simulink model "nms_sim_2D_cost"  (R2024b)
settings: Solver=ode15s  StartTime=0.0  StopTime=t_sim  MaxStep=dt_max  EnableMultiTasking=on
values from neighbouring files (symbols this model uses):
  a_BFSH = param_ctrl(35)*1    [setCtrlPar_optim_CPGreflex2001_2D.m]
  a_GAS = param_ctrl(37)*1    [setCtrlPar_optim_CPGreflex2001_2D.m]
  a_GLU = param_ctrl(31)*1    [setCtrlPar_optim_CPGreflex2001_2D.m]
  a_HAM = param_ctrl(33)*1    [setCtrlPar_optim_CPGreflex2001_2D.m]
  a_HFL = param_ctrl(32)*1    [setCtrlPar_optim_CPGreflex2001_2D.m]
  a_RF = param_ctrl(34)*1    [setCtrlPar_optim_CPGreflex2001_2D.m]
  a_SOL = param_ctrl(38)*1    [setCtrlPar_optim_CPGreflex2001_2D.m]
  a_TA = param_ctrl(39)*1    [setCtrlPar_optim_CPGreflex2001_2D.m]
  a_VAS = param_ctrl(36)*1    [setCtrlPar_optim_CPGreflex2001_2D.m]
  ai = param_ctrl(96)*2.0    [setCtrlPar_optim_CPGreflex2001_2D.m]
  b_BFSH = param_ctrl(52)*.51    [setCtrlPar_optim_CPGreflex2001_2D.m]
  b_BFSHGAS = param_ctrl(55)*.51    [setCtrlPar_optim_CPGreflex2001_2D.m]
  b_BFSHHAM = param_ctrl(54)*.51    [setCtrlPar_optim_CPGreflex2001_2D.m]
  b_BFSHVAS = param_ctrl(53)*.51    [setCtrlPar_optim_CPGreflex2001_2D.m]
  b_GAS = param_ctrl(59)*.51    [setCtrlPar_optim_CPGreflex2001_2D.m]
  b_GASBFSH = param_ctrl(60)*.51    [setCtrlPar_optim_CPGreflex2001_2D.m]
  b_GASSOL = param_ctrl(61)*.51    [setCtrlPar_optim_CPGreflex2001_2D.m]
  b_GLU = param_ctrl(40)*.51    [setCtrlPar_optim_CPGreflex2001_2D.m]
  b_GLUHAM = param_ctrl(42)*.51    [setCtrlPar_optim_CPGreflex2001_2D.m]
  b_GLUHFL = param_ctrl(41)*.51    [setCtrlPar_optim_CPGreflex2001_2D.m]
  b_HAM = param_ctrl(46)*.51    [setCtrlPar_optim_CPGreflex2001_2D.m]
  b_HAMBFSH = param_ctrl(48)*.51    [setCtrlPar_optim_CPGreflex2001_2D.m]
  b_HAMGLU = param_ctrl(47)*.51    [setCtrlPar_optim_CPGreflex2001_2D.m]
  b_HFL = param_ctrl(43)*.51    [setCtrlPar_optim_CPGreflex2001_2D.m]
  b_HFLGLU = param_ctrl(44)*.51    [setCtrlPar_optim_CPGreflex2001_2D.m]
  b_HFLRF = param_ctrl(45)*.51    [setCtrlPar_optim_CPGreflex2001_2D.m]
  b_RF = param_ctrl(49)*.51    [setCtrlPar_optim_CPGreflex2001_2D.m]
  b_RFHFL = param_ctrl(50)*.51    [setCtrlPar_optim_CPGreflex2001_2D.m]
  b_RFVAS = param_ctrl(51)*.51    [setCtrlPar_optim_CPGreflex2001_2D.m]
  b_SOL = param_ctrl(62)*.51    [setCtrlPar_optim_CPGreflex2001_2D.m]
  b_SOLGAS = param_ctrl(64)*.51    [setCtrlPar_optim_CPGreflex2001_2D.m]
  b_SOLTA = param_ctrl(63)*.51    [setCtrlPar_optim_CPGreflex2001_2D.m]
  b_TA = param_ctrl(65)*.51    [setCtrlPar_optim_CPGreflex2001_2D.m]
  b_TASOL = param_ctrl(66)*.51    [setCtrlPar_optim_CPGreflex2001_2D.m]
  b_VAS = param_ctrl(56)*.51    [setCtrlPar_optim_CPGreflex2001_2D.m]
  b_VASBFSH = param_ctrl(57)*.51    [setCtrlPar_optim_CPGreflex2001_2D.m]
  b_VASRF = param_ctrl(58)*.51    [setCtrlPar_optim_CPGreflex2001_2D.m]
  bias = param_ctrl(97)*2.5    [setCtrlPar_optim_CPGreflex2001_2D.m]
  c = 0.05    [nms_MS_2D_scaled.m]
  c_jointstop = 0.3 / (pi/180)    (= 17.1887338539)    [nms_MS_2D_scaled.m]
  D12_F = 0.16    *scaleL_JPhys    [nms_MechInit_2D_scaleSkel.m]
  D12_S = 0.2460	*sub_height    [nms_MechInit_2D_scaleSkel.m]
  D12_T = 0.2450  *sub_height    [nms_MechInit_2D_scaleSkel.m]
  D12y_F = 0.039  *sub_height    [nms_MechInit_2D_scaleSkel.m]
  D12z_HAT = 0.1    [nms_MS_2D_scaled.m]
  D13_F = 0.20    *scaleL_JPhys    [nms_MechInit_2D_scaleSkel.m]
  D1G_F = 0.14    *scaleL_JPhys    [nms_MechInit_2D_scaleSkel.m]
  D1G_HAT = 0.35  *scaleL_JPhys    [nms_MechInit_2D_scaleSkel.m]
  D1G_S = (0.3 - D12y_F/4)	*scaleL_JPhys    [nms_MechInit_2D_scaleSkel.m]
  D1G_T = (0.3 - D12y_F/4)	*scaleL_JPhys    [nms_MechInit_2D_scaleSkel.m]
  D1Gy_F = D12y_F*D1G_F/D12_F    (= 0.07)    [nms_MechInit_2D_scaleSkel.m]
  d_BFSH = param_ctrl(26)*1    [setCtrlPar_optim_CPGreflex2001_2D.m]
  d_GAS = param_ctrl(28)*1    [setCtrlPar_optim_CPGreflex2001_2D.m]
  d_GLU = param_ctrl(22)*1    [setCtrlPar_optim_CPGreflex2001_2D.m]
  d_HAM = param_ctrl(24)*1    [setCtrlPar_optim_CPGreflex2001_2D.m]
  d_HFL = param_ctrl(23)*1    [setCtrlPar_optim_CPGreflex2001_2D.m]
  d_RF = param_ctrl(25)*1    [setCtrlPar_optim_CPGreflex2001_2D.m]
  d_SOL = param_ctrl(29)*1    [setCtrlPar_optim_CPGreflex2001_2D.m]
  d_TA = param_ctrl(30)*1    [setCtrlPar_optim_CPGreflex2001_2D.m]
  d_VAS = param_ctrl(27)*1    [setCtrlPar_optim_CPGreflex2001_2D.m]
  DeltaThRef = 5e-3    (= 0.005)    [nms_MS_2D_scaled.m]
  dloptBFSH = 3.0    (= 3)    [setCtrlPar_optim_CPGreflex2001_2D.m]
  dloptGAS = 3.0    (= 3)    [setCtrlPar_optim_CPGreflex2001_2D.m]
  dloptGLU = 3.0    (= 3)    [setCtrlPar_optim_CPGreflex2001_2D.m]
  dloptHAM = 3.0    (= 3)    [setCtrlPar_optim_CPGreflex2001_2D.m]
  dloptHFL = 3.0    (= 3)    [setCtrlPar_optim_CPGreflex2001_2D.m]
  dloptRF = 3.0    (= 3)    [setCtrlPar_optim_CPGreflex2001_2D.m]
  dloptSOL = 3.0    (= 3)    [setCtrlPar_optim_CPGreflex2001_2D.m]
  dloptTA = 3.0    (= 3)    [setCtrlPar_optim_CPGreflex2001_2D.m]
  dloptVAS = 3.0    (= 3)    [setCtrlPar_optim_CPGreflex2001_2D.m]
  ec_BFSH = param_ctrl(80)*0.15    [setCtrlPar_optim_CPGreflex2001_2D.m]
  ec_GAS = param_ctrl(82)*0.15    [setCtrlPar_optim_CPGreflex2001_2D.m]
  ec_GLU = param_ctrl(76)*0.15    [setCtrlPar_optim_CPGreflex2001_2D.m]
  ec_HAM = param_ctrl(78)*0.15    [setCtrlPar_optim_CPGreflex2001_2D.m]
  ec_HFL = param_ctrl(77)*0.15    [setCtrlPar_optim_CPGreflex2001_2D.m]
  ec_RF = param_ctrl(79)*0.15    [setCtrlPar_optim_CPGreflex2001_2D.m]
  ec_TA = param_ctrl(84)*0.15    [setCtrlPar_optim_CPGreflex2001_2D.m]
  ec_VAS = param_ctrl(81)*0.15    [setCtrlPar_optim_CPGreflex2001_2D.m]
  eref = 0.04    [nms_MS_2D_scaled.m]
  eref_GAS = 0.1    [nms_MS_2D_scaled.m]
  eref_SOL = 0.1    [nms_MS_2D_scaled.m]
  es_BFSH = param_ctrl(89)*0.15    [setCtrlPar_optim_CPGreflex2001_2D.m]
  es_GAS = param_ctrl(91)*0.15    [setCtrlPar_optim_CPGreflex2001_2D.m]
  es_GLU = param_ctrl(85)*0.15    [setCtrlPar_optim_CPGreflex2001_2D.m]
  es_HAM = param_ctrl(87)*0.15    [setCtrlPar_optim_CPGreflex2001_2D.m]
  es_HFL = param_ctrl(86)*0.15    [setCtrlPar_optim_CPGreflex2001_2D.m]
  es_RF = param_ctrl(88)*0.15    [setCtrlPar_optim_CPGreflex2001_2D.m]
  es_TA = param_ctrl(93)*0.15    [setCtrlPar_optim_CPGreflex2001_2D.m]
  es_VAS = param_ctrl(90)*0.15    [setCtrlPar_optim_CPGreflex2001_2D.m]
  FmaxBFSH = 350    [nms_MS_2D_scaled.m]
  FmaxGAS = 2000    [nms_MS_2D_scaled.m]
  FmaxGLU = 4000    [nms_MS_2D_scaled.m]
  FmaxHAM = 2000    [nms_MS_2D_scaled.m]
  FmaxHFL = 2000    [nms_MS_2D_scaled.m]
  FmaxRF = 850    [nms_MS_2D_scaled.m]
  FmaxSOL = 4000    [nms_MS_2D_scaled.m]
  FmaxTA = 800    [nms_MS_2D_scaled.m]
  FmaxVAS = 5000    [nms_MS_2D_scaled.m]
  g = 9.81    [nms_MS_2D_scaled.m]
  gamma_4 = param_ctrl(11) * 1.7    [setCtrlPar_optim_CPGreflexsynergy2023_2D.m]
  h_BFSH = param_ctrl(71)*.1    [setCtrlPar_optim_CPGreflex2001_2D.m]
  h_GAS = param_ctrl(73)*.1    [setCtrlPar_optim_CPGreflex2001_2D.m]
  h_GLU = param_ctrl(67)*.1    [setCtrlPar_optim_CPGreflex2001_2D.m]
  h_HAM = param_ctrl(69)*.1    [setCtrlPar_optim_CPGreflex2001_2D.m]
  h_HFL = param_ctrl(68)*.1    [setCtrlPar_optim_CPGreflex2001_2D.m]
  h_RF = param_ctrl(70)*.1    [setCtrlPar_optim_CPGreflex2001_2D.m]
  h_SOL = param_ctrl(74)*.1    [setCtrlPar_optim_CPGreflex2001_2D.m]
  h_TA = param_ctrl(75)*.1    [setCtrlPar_optim_CPGreflex2001_2D.m]
  h_VAS = param_ctrl(72)*.1    [setCtrlPar_optim_CPGreflex2001_2D.m]
  HLCtrlPar = [theta_tgt l_clr alpha_tgt alpha_cd alpha_cv]    [setCtrlPar_optim_reflex2015_2D.m]
  In_F = 0.005    *scaleM*scaleL_JPhys^2    [nms_MechInit_2D_scaleSkel.m]
  In_HAT = 2.5    *scaleM*scaleL_JPhys^2    [nms_MechInit_2D_scaleSkel.m]
  In_S = 0.05     *scaleM*scaleL_JPhys^2    [nms_MechInit_2D_scaleSkel.m]
  In_T = 0.15     *scaleM*scaleL_JPhys^2    [nms_MechInit_2D_scaleSkel.m]
  init_exc = 0.01    [setInitPar_optim_2D.m]
  init_fm = 0.01    [setInitPar_optim_2D.m]
  init_lce = 1    [setInitPar_optim_2D.m]
  init_LCPG = param_ctrl(12) * 0.01    [setCtrlPar_optim_CPGreflexsynergy2023_2D.m]
  init_LStance = 1    [setInitPar_optim_2D.m]
  init_N1 = osc_signal1(phi_off_osc_ind)    [setCtrlPar_optim_CPGreflex2001_2D.m]
  ... (+441 more)
undefined symbols (not defined in the file or in its folder): cost_act_exponent, cost_v_tgt, flag_controller, Newton, nStep_obj, nStep_startKin, Raphson, sgn, SSW_kin, terrain_slope_angle, v_plateS1, X, Y, Z
libraries: nesl_utility x94, sm_lib x90, simulink x28, simulink_extras x12
(part 1 of 20)
settings Model: SimulationMode=accelerator  Creator=smsong  LastModifiedBy=tonvi
settings SolverCC: ZeroCrossControl=DisableAll  AlgebraicLoopSolver=TrustRegion
settings DataIOCC: LimitDataPoints=on  SaveFormat=Array  SaveOutput=off  SignalLogging=off  DSMLogging=off  SaveTime=off
settings OptimizationCC: BooleanDataType=off  ReuseModelBlockBuffer=off  LifeSpan=inf
settings DebuggingCC: UnconnectedInputMsg=warning  UnconnectedOutputMsg=warning  UnconnectedLineMsg=warning  SFUnexpectedBacktrackingDiag=warning  SFNoUnconditionalDefaultTransitionDiag=warning  SFExecutionAtInitializationDiag=none  ArithmeticOperatorsInVariantConditions=warning
settings HardwareCC: ProdBitPerPointer=32  ProdBitPerSizeT=32  ProdBitPerPtrDiffT=32  ProdLargestAtomicFloat=None  ProdIntDivRoundTo=Undefined  ProdEndianess=Unspecified  ProdWordSize=32  ProdHWDeviceType=32-bit Generic
settings ModelReferenceCC: EnableRefExpFcnMdlSchedulingChecks=on  PropagateSignalLabelsOutOfModel=off
settings SFSimCC: SimUseLocalCustomCode=off  CustomCodeUndefinedFunction=UseInterfaceOnly
settings RTWCC: RTWUseLocalCustomCode=off  GPUComputeCapability=3.5
settings CodeAppCC: StateflowObjectComments=on
settings GRTTargetCC: TargetLangStandard=C89/C90 (ANSI)
settings ConfigComp: CovMetricSettings=dw  CovSaveCumulativeToWorkspaceVar=on  CovSaveSingleToWorkspaceVar=on  CovExternalEMLEnable=off
settings SimscapeCC: SimscapeNormalizeSystem=off
settings ConfigurationSet: Description=SimMechanics 2G
settings ExplorerConfigSet: InternalSimMechanicsExplorerSettings="<ExplorerConfiguration><canonicalview>planar_xy</canonicalview><AnimationSetting><BasePlaybackSpeed>1.0</BasePlaybackSpeed><PlaybackSpeedFactor>1.0</PlaybackSpeedFactor></AnimationSetting><TilePanel><TileInfo><Tiles Columns=\"1\" Count=\"1\" Rows=\"1\"><Column Weight=\"1\"/><Row Weight=\"1\"/><Tile Height=\"1\" Width=\"1\" X=\"0\" Y=\"0\"/></Tiles></TileInfo><SceneInfo><SceneViewer><BGColor><R>1</R><G>1</G><B>1</B></BGColor><Camera><DoPerspective>off</DoPerspective><Position><X>-0.261050130897375665</X><Y>1.42717715276589785</Y><Z>30.2910165948773908</Z></Position><Center><X>-0.261050130897375665</X><Y>1.42717715276589785</Y><Z>-2.94192883387722759e-08</Z></Center><Up><X>0</X><Y>1</Y><Z>0</Z></Up><ViewLimDist>1</ViewLimDist><YLim>2.31502487225703657</YLim><XLim>2.56039617208151515</XLim></Camera></SceneViewer></SceneInfo></TilePanel><MechEditorPanel><Cameras/><GfxPanelCameraMap/><VideoCreator><PlaybackSpeedRatio>1.0</PlaybackSpeedRatio><FrameRate>30</FrameRate><VideoFormat>Motion JPEG AVI</VideoFormat><FrameSize>auto</FrameSize></VideoCreator></MechEditorPanel></ExplorerConfiguration>"

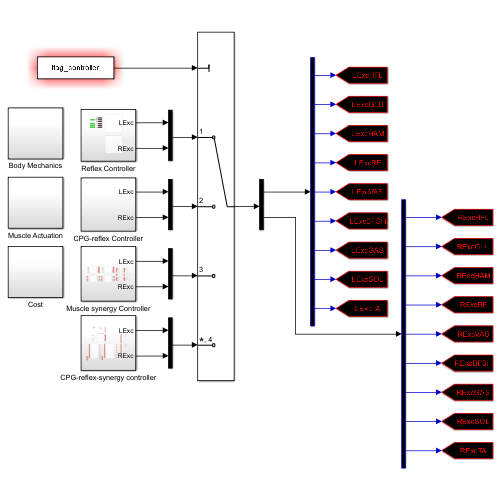
[thumbnail: Simulink's stored preview of the top-level diagram]
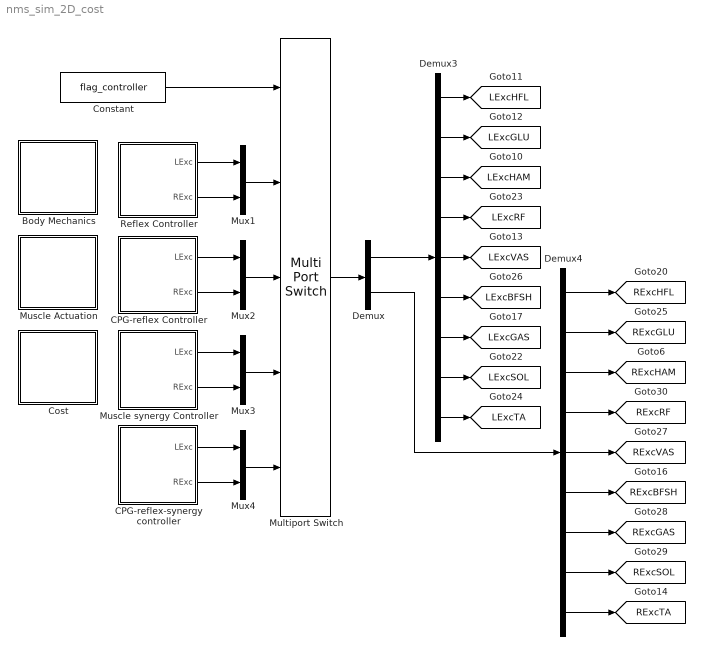
== system nms_sim_2D_cost ==
  Body Mechanics : Subsystem
  CPG-reflex Controller : Subsystem
  CPG-reflex-synergy controller : Subsystem
  Constant : Constant  Value=flag_controller
  Cost : Subsystem
  Demux : Demux  Outputs=2
  Demux3 : Demux  Outputs=9
  Demux4 : Demux  Outputs=9
  Multiport Switch : MultiPortSwitch  Inputs=4  SaturateOnIntegerOverflow=off  InputSameDT=off
  Muscle Actuation : Subsystem
  Muscle synergy Controller : Subsystem
  Mux{1..4} (4 alike) : Mux  Inputs=2
  Reflex Controller : Subsystem
  tag scope: LExcBFSH=global, LExcGAS=global, LExcGLU=global, LExcHAM=global, LExcHFL=global, LExcRF=global, LExcSOL=global, LExcTA=global, LExcVAS=global, RExcBFSH=global, RExcGAS=global, RExcGLU=global, RExcHAM=global, RExcHFL=global, RExcRF=global, RExcSOL=global, RExcTA=global, RExcVAS=global
  wires:
  Demux3/9 -> [LExcTA]
  Demux/1 -> Demux3/1
  Demux3/4 -> [LExcRF]
  Demux3/6 -> [LExcBFSH]
  Demux3/1 -> [LExcHFL]
  Demux3/8 -> [LExcSOL]
  Demux3/3 -> [LExcHAM]
  Demux3/7 -> [LExcGAS]
  Demux3/5 -> [LExcVAS]
  Demux3/2 -> [LExcGLU]
  Demux/2 -> Demux4/1
  Demux4/7 -> [RExcGAS]
  Demux4/8 -> [RExcSOL]
  Demux4/5 -> [RExcVAS]
  Demux4/2 -> [RExcGLU]
  Demux4/4 -> [RExcRF]
  Demux4/3 -> [RExcHAM]
  Demux4/1 -> [RExcHFL]
  Demux4/6 -> [RExcBFSH]
  Demux4/9 -> [RExcTA]
  Constant/1 -> Multiport Switch/1
  Reflex Controller/1(LExc) -> Mux1/1
  Reflex Controller/2(RExc) -> Mux1/2
  CPG-reflex-synergy controller/2(RExc) -> Mux4/2
  CPG-reflex-synergy controller/1(LExc) -> Mux4/1
  Multiport Switch/1 -> Demux/1
  Mux1/1 -> Multiport Switch/2
  Mux4/1 -> Multiport Switch/5
  Muscle synergy Controller/1(LExc) -> Mux3/1
  Muscle synergy Controller/2(RExc) -> Mux3/2
  Mux2/1 -> Multiport Switch/3
  Mux3/1 -> Multiport Switch/4
  CPG-reflex Controller/1(LExc) -> Mux2/1
  CPG-reflex Controller/2(RExc) -> Mux2/2

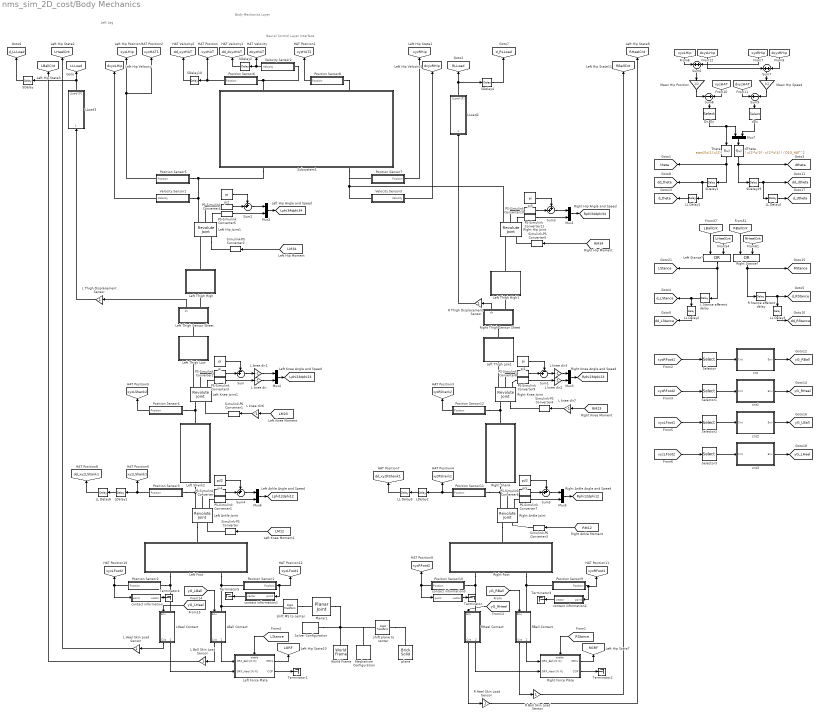
== system nms_sim_2D_cost/Body Mechanics ==
  note: Body Mechanics Layer
  note: Left Leg
  note: Neural Control Layer Interface
  " Mean Hip Speed" : Gain  Gain=1/2
  "Dx, Dy" : Selector  InputPortWidth=3  IndexOptions=Index vector (dialog)  Indices=[1 2]  OutputSizes=1
  L Ball Skin Load Sensor : Gain
  L Heel Skin Load Sensor : Gain
  L Stance afferent delay : TransportDelay  DelayTime=MidDelay  InitialOutput=init_LStance
  L Thigh Displacement  Sensor : Gain
  L knee dir{,1..3,6..7} (6 alike) : Gain  Gain=-1
  LBall Contact : Subsystem
  LDelay1 : TransportDelay  DelayTime=LongDelay  InitialOutput=init_xyzLShank
  LDelay2 : TransportDelay  DelayTime=LongDelay  InitialOutput=init_xyzRShank
  LHeel Contact : Subsystem
  LL Delay1 : TransportDelay  DelayTime=LongLoopDelay  InitialOutput=init_theta
  LL Delay2 : TransportDelay  DelayTime=LongLoopDelay  InitialOutput=init_LStance
  LL Delay3 : TransportDelay  DelayTime=LongLoopDelay  InitialOutput=init_RStance
  LL Delay4 : TransportDelay  DelayTime=LongLoopDelay
  LL Delay5 : TransportDelay  DelayTime=LongLoopDelay  InitialOutput=init_xyzRShank
  LL Delay6 : TransportDelay  DelayTime=LongLoopDelay  InitialOutput=init_xyzLShank
  LLoad2 : Subsystem
  LLoad3 : Subsystem
  Left Ankle Joint : sm_lib/Joints/Revolute Joint  JointMode=Normal  CompositeWrenchDir=FollowerOnBase  CompositeWrenchFrame=BaseFrame  SenseConstraintForce=off  SenseConstraintTorque=off  SenseTotalForce=off  SenseTotalTorque=off  PositionTargetSpecify=on  PositionTargetPriority=High  PositionTargetValue=Lphi120-pi/2  PositionTargetValueUnits=rad  VelocityTargetSpecify=on  VelocityTargetPriority=High  VelocityTargetValue=0  VelocityTargetValueUnits=rad/s  EquilibriumPosition=0  EquilibriumPositionUnits=deg  SpringStiffness=0  SpringStiffnessUnits=N*m/deg  DampingCoefficient=0  DampingCoefficientUnits=N*m/(deg/s)  LowerLimitSpecify=off  LowerLimitBound=-90  LowerLimitBoundUnits=deg  LowerLimitStiffness=1e4  LowerLimitStiffnessUnits=N*m/deg  LowerLimitDamping=10  LowerLimitDampingUnits=N*m/(deg/s)  LowerLimitTransitionRegionWidth=0.1  LowerLimitTransitionRegionWidthUnits=deg  UpperLimitSpecify=off  UpperLimitBound=90  UpperLimitBoundUnits=deg  UpperLimitStiffness=1e4  UpperLimitStiffnessUnits=N*m/deg  UpperLimitDamping=10  UpperLimitDampingUnits=N*m/(deg/s)  UpperLimitTransitionRegionWidth=0.1  UpperLimitTransitionRegionWidthUnits=deg  TorqueActuationMode=InputTorque  MotionActuationMode=ComputedMotion  SensePosition=on  SenseVelocity=on  SenseAcceleration=off  SenseTorqueForce=off  SenseLowerLimitTorqueForce=off  SenseUpperLimitTorqueForce=off
  Left Hip Joint1 : sm_lib/Joints/Revolute Joint  JointMode=Normal  CompositeWrenchDir=FollowerOnBase  CompositeWrenchFrame=BaseFrame  SenseConstraintForce=off  SenseConstraintTorque=off  SenseTotalForce=off  SenseTotalTorque=off  PositionTargetSpecify=on  PositionTargetPriority=High  PositionTargetValue=Lphi340-pi  PositionTargetValueUnits=rad  VelocityTargetSpecify=on  VelocityTargetPriority=High  VelocityTargetValue=0  VelocityTargetValueUnits=rad/s  EquilibriumPosition=0  EquilibriumPositionUnits=deg  SpringStiffness=0  SpringStiffnessUnits=N*m/deg  DampingCoefficient=0  DampingCoefficientUnits=N*m/(deg/s)  LowerLimitSpecify=off  LowerLimitBound=-90  LowerLimitBoundUnits=deg  LowerLimitStiffness=1e4  LowerLimitStiffnessUnits=N*m/deg  LowerLimitDamping=10  LowerLimitDampingUnits=N*m/(deg/s)  LowerLimitTransitionRegionWidth=0.1  LowerLimitTransitionRegionWidthUnits=deg  UpperLimitSpecify=off  UpperLimitBound=90  UpperLimitBoundUnits=deg  UpperLimitStiffness=1e4  UpperLimitStiffnessUnits=N*m/deg  UpperLimitDamping=10  UpperLimitDampingUnits=N*m/(deg/s)  UpperLimitTransitionRegionWidth=0.1  UpperLimitTransitionRegionWidthUnits=deg  TorqueActuationMode=InputTorque  MotionActuationMode=ComputedMotion  SensePosition=on  SenseVelocity=on  SenseAcceleration=off  SenseTorqueForce=off  SenseLowerLimitTorqueForce=off  SenseUpperLimitTorqueForce=off
  Left Knee Joint1 : sm_lib/Joints/Revolute Joint  JointMode=Normal  CompositeWrenchDir=FollowerOnBase  CompositeWrenchFrame=BaseFrame  SenseConstraintForce=off  SenseConstraintTorque=off  SenseTotalForce=off  SenseTotalTorque=off  PositionTargetSpecify=on  PositionTargetPriority=High  PositionTargetValue=pi-Lphi230  PositionTargetValueUnits=rad  VelocityTargetSpecify=on  VelocityTargetPriority=High  VelocityTargetValue=0  VelocityTargetValueUnits=rad/s  EquilibriumPosition=0  EquilibriumPositionUnits=deg  SpringStiffness=0  SpringStiffnessUnits=N*m/deg  DampingCoefficient=0  DampingCoefficientUnits=N*m/(deg/s)  LowerLimitSpecify=off  LowerLimitBound=-90  LowerLimitBoundUnits=deg  LowerLimitStiffness=1e4  LowerLimitStiffnessUnits=N*m/deg  LowerLimitDamping=10  LowerLimitDampingUnits=N*m/(deg/s)  LowerLimitTransitionRegionWidth=0.1  LowerLimitTransitionRegionWidthUnits=deg  UpperLimitSpecify=off  UpperLimitBound=90  UpperLimitBoundUnits=deg  UpperLimitStiffness=1e4  UpperLimitStiffnessUnits=N*m/deg  UpperLimitDamping=10  UpperLimitDampingUnits=N*m/(deg/s)  UpperLimitTransitionRegionWidth=0.1  UpperLimitTransitionRegionWidthUnits=deg  TorqueActuationMode=InputTorque  MotionActuationMode=ComputedMotion  SensePosition=on  SenseVelocity=on  SenseAcceleration=off  SenseTorqueForce=off  SenseLowerLimitTorqueForce=off  SenseUpperLimitTorqueForce=off
  Left Foot : Subsystem
  Left Force Plate : Subsystem  TreatAsAtomicUnit=on
  Left Shank2 : Subsystem
  Left Stance? : Logic  Operator=OR  AllPortsSameDT=off
  Left Thigh Sensor Sheet : Subsystem
  Left Thigh High : Subsystem
  Left Thigh High1 : Subsystem
  Left Thigh Low : Subsystem
  Left Thigh Low1 : Subsystem
  Mean Hip Position : Gain  Gain=1/2
  Mechanism Configuration : sm_lib/Utilities/Mechanism Configuration  UniformGravity=Constant  GravityVector=[0 -g 0]  GravityVectorUnits=m/s^2  LinearizationDelta=0.001  JointModeTransitionNonlinearIterations=2
  Mux{1..7} (7 alike) : Mux  Inputs=2
  PS-Simulink Converter{,2,4,6,8,10} (6 alike) : nesl_utility/PS-Simulink Converter  PhysicalDomain=network_engine_domain  SubClassName=ps_output  LeftPortType=input  RightPortType=output  PseudoPeriodic=off  Frequencies=[]  VectorFormat=1-D array  Unit=rad  AffineConversion=off
  PS-Simulink Converter{1,3,5,7,9,11} (6 alike) : nesl_utility/PS-Simulink Converter  PhysicalDomain=network_engine_domain  SubClassName=ps_output  LeftPortType=input  RightPortType=output  PseudoPeriodic=off  Frequencies=[]  VectorFormat=1-D array  Unit=rad/s  AffineConversion=off
  Planar1 : sm_lib/Joints/Planar Joint  JointMode=Normal  CompositeWrenchDir=FollowerOnBase  CompositeWrenchFrame=BaseFrame  SenseConstraintForce=off  SenseConstraintTorque=off  SenseTotalForce=off  SenseTotalTorque=off  PxPositionTargetSpecify=on  PxPositionTargetPriority=High  PxPositionTargetValue=x0  PxPositionTargetValueUnits=m  PxVelocityTargetSpecify=on  PxVelocityTargetPriority=High  PxVelocityTargetValue=vx0  PxVelocityTargetValueUnits=m/s  PxEquilibriumPosition=0  PxEquilibriumPositionUnits=m  PxSpringStiffness=0  PxSpringStiffnessUnits=N/m  PxDampingCoefficient=0  PxDampingCoefficientUnits=N/(m/s)  PxLowerLimitSpecify=off  PxLowerLimitBound=-1  PxLowerLimitBoundUnits=m  PxLowerLimitStiffness=1e6  PxLowerLimitStiffnessUnits=N/m  PxLowerLimitDamping=1e3  PxLowerLimitDampingUnits=N/(m/s)  PxLowerLimitTransitionRegionWidth=1e-4  PxLowerLimitTransitionRegionWidthUnits=m  PxUpperLimitSpecify=off  PxUpperLimitBound=1  PxUpperLimitBoundUnits=m  PxUpperLimitStiffness=1e6  PxUpperLimitStiffnessUnits=N/m  PxUpperLimitDamping=1e3  PxUpperLimitDampingUnits=N/(m/s)  PxUpperLimitTransitionRegionWidth=1e-4  PxUpperLimitTransitionRegionWidthUnits=m  PxTorqueActuationMode=NoTorque  PxMotionActuationMode=ComputedMotion  PxSensePosition=off  PxSenseVelocity=off  PxSenseAcceleration=off  PxSenseTorqueForce=off  PxSenseLowerLimitTorqueForce=off  PxSenseUpperLimitTorqueForce=off  PyPositionTargetSpecify=on  PyPositionTargetPriority=High  PyPositionTargetValue=y0  PyPositionTargetValueUnits=m  PyVelocityTargetSpecify=on  PyVelocityTargetPriority=High  PyVelocityTargetValue=0  PyVelocityTargetValueUnits=m/s  PyEquilibriumPosition=0  PyEquilibriumPositionUnits=m  PySpringStiffness=0  PySpringStiffnessUnits=N/m  PyDampingCoefficient=0  PyDampingCoefficientUnits=N/(m/s)  PyLowerLimitSpecify=off  PyLowerLimitBound=-1  PyLowerLimitBoundUnits=m  PyLowerLimitStiffness=1e6  PyLowerLimitStiffnessUnits=N/m  PyLowerLimitDamping=1e3  PyLowerLimitDampingUnits=N/(m/s)  PyLowerLimitTransitionRegionWidth=1e-4  PyLowerLimitTransitionRegionWidthUnits=m  PyUpperLimitSpecify=off  PyUpperLimitBound=1  PyUpperLimitBoundUnits=m  PyUpperLimitStiffness=1e6  PyUpperLimitStiffnessUnits=N/m  PyUpperLimitDamping=1e3  PyUpperLimitDampingUnits=N/(m/s)  PyUpperLimitTransitionRegionWidth=1e-4  PyUpperLimitTransitionRegionWidthUnits=m  PyTorqueActuationMode=NoTorque  PyMotionActuationMode=ComputedMotion  PySensePosition=off  PySenseVelocity=off  PySenseAcceleration=off  PySenseTorqueForce=off  PySenseLowerLimitTorqueForce=off  PySenseUpperLimitTorqueForce=off  RzPositionTargetSpecify=on  RzPositionTargetPriority=High  RzPositionTargetValue=phi0  RzPositionTargetValueUnits=rad  RzVelocityTargetSpecify=on  RzVelocityTargetPriority=High  RzVelocityTargetValue=0  RzVelocityTargetValueUnits=rad/s  RzEquilibriumPosition=0  RzEquilibriumPositionUnits=deg  RzSpringStiffness=0  RzSpringStiffnessUnits=N*m/deg  RzDampingCoefficient=0  RzDampingCoefficientUnits=N*m/(deg/s)  RzLowerLimitSpecify=off  RzLowerLimitBound=-90  RzLowerLimitBoundUnits=deg  RzLowerLimitStiffness=1e4  RzLowerLimitStiffnessUnits=N*m/deg  RzLowerLimitDamping=10  RzLowerLimitDampingUnits=N*m/(deg/s)  RzLowerLimitTransitionRegionWidth=0.1  RzLowerLimitTransitionRegionWidthUnits=deg  RzUpperLimitSpecify=off  RzUpperLimitBound=90  RzUpperLimitBoundUnits=deg  RzUpperLimitStiffness=1e4  RzUpperLimitStiffnessUnits=N*m/deg  RzUpperLimitDamping=10  RzUpperLimitDampingUnits=N*m/(deg/s)  RzUpperLimitTransitionRegionWidth=0.1  RzUpperLimitTransitionRegionWidthUnits=deg  RzTorqueActuationMode=NoTorque  RzMotionActuationMode=ComputedMotion  RzSensePosition=off  RzSenseVelocity=off  RzSenseAcceleration=off  RzSenseTorqueForce=off  RzSenseLowerLimitTorqueForce=off  RzSenseUpperLimitTorqueForce=off
  Position Sensor1 : Subsystem
  Position Sensor10 : Subsystem
  Position Sensor11 : Subsystem
  Position Sensor12 : Subsystem
  Position Sensor2 : Subsystem
  Position Sensor3 : Subsystem
  Position Sensor4 : Subsystem
  Position Sensor5 : Subsystem
  Position Sensor6 : Subsystem
  Position Sensor7 : Subsystem
  Position Sensor8 : Subsystem
  Position Sensor9 : Subsystem
  R Ball Skin Load Sensor : Gain
  R Heel Skin Load Sensor : Gain
  R Stance afferent delay : TransportDelay  DelayTime=MidDelay  InitialOutput=init_RStance
  R Thigh Displacement  Sensor : Gain
  RBall Contact : Subsystem
  RHeel Contact : Subsystem
  Right Ankle Joint : sm_lib/Joints/Revolute Joint  JointMode=Normal  CompositeWrenchDir=FollowerOnBase  CompositeWrenchFrame=BaseFrame  SenseConstraintForce=off  SenseConstraintTorque=off  SenseTotalForce=off  SenseTotalTorque=off  PositionTargetSpecify=on  PositionTargetPriority=High  PositionTargetValue=Rphi120-pi/2  PositionTargetValueUnits=rad  VelocityTargetSpecify=on  VelocityTargetPriority=High  VelocityTargetValue=0  VelocityTargetValueUnits=rad/s  EquilibriumPosition=0  EquilibriumPositionUnits=deg  SpringStiffness=0  SpringStiffnessUnits=N*m/deg  DampingCoefficient=0  DampingCoefficientUnits=N*m/(deg/s)  LowerLimitSpecify=off  LowerLimitBound=-90  LowerLimitBoundUnits=deg  LowerLimitStiffness=1e4  LowerLimitStiffnessUnits=N*m/deg  LowerLimitDamping=10  LowerLimitDampingUnits=N*m/(deg/s)  LowerLimitTransitionRegionWidth=0.1  LowerLimitTransitionRegionWidthUnits=deg  UpperLimitSpecify=off  UpperLimitBound=90  UpperLimitBoundUnits=deg  UpperLimitStiffness=1e4  UpperLimitStiffnessUnits=N*m/deg  UpperLimitDamping=10  UpperLimitDampingUnits=N*m/(deg/s)  UpperLimitTransitionRegionWidth=0.1  UpperLimitTransitionRegionWidthUnits=deg  TorqueActuationMode=InputTorque  MotionActuationMode=ComputedMotion  SensePosition=on  SenseVelocity=on  SenseAcceleration=off  SenseTorqueForce=off  SenseLowerLimitTorqueForce=off  SenseUpperLimitTorqueForce=off
  Right Hip Joint : sm_lib/Joints/Revolute Joint  JointMode=Normal  CompositeWrenchDir=FollowerOnBase  CompositeWrenchFrame=BaseFrame  SenseConstraintForce=off  SenseConstraintTorque=off  SenseTotalForce=off  SenseTotalTorque=off  PositionTargetSpecify=on  PositionTargetPriority=High  PositionTargetValue=Rphi340-pi  PositionTargetValueUnits=rad  VelocityTargetSpecify=on  VelocityTargetPriority=High  VelocityTargetValue=0  VelocityTargetValueUnits=rad/s  EquilibriumPosition=0  EquilibriumPositionUnits=deg  SpringStiffness=0  SpringStiffnessUnits=N*m/deg  DampingCoefficient=0  DampingCoefficientUnits=N*m/(deg/s)  LowerLimitSpecify=off  LowerLimitBound=-90  LowerLimitBoundUnits=deg  LowerLimitStiffness=1e4  LowerLimitStiffnessUnits=N*m/deg  LowerLimitDamping=10  LowerLimitDampingUnits=N*m/(deg/s)  LowerLimitTransitionRegionWidth=0.1  LowerLimitTransitionRegionWidthUnits=deg  UpperLimitSpecify=off  UpperLimitBound=90  UpperLimitBoundUnits=deg  UpperLimitStiffness=1e4  UpperLimitStiffnessUnits=N*m/deg  UpperLimitDamping=10  UpperLimitDampingUnits=N*m/(deg/s)  UpperLimitTransitionRegionWidth=0.1  UpperLimitTransitionRegionWidthUnits=deg  TorqueActuationMode=InputTorque  MotionActuationMode=ComputedMotion  SensePosition=on  SenseVelocity=on  SenseAcceleration=off  SenseTorqueForce=off  SenseLowerLimitTorqueForce=off  SenseUpperLimitTorqueForce=off
  Right Knee Joint : sm_lib/Joints/Revolute Joint  JointMode=Normal  CompositeWrenchDir=FollowerOnBase  CompositeWrenchFrame=BaseFrame  SenseConstraintForce=off  SenseConstraintTorque=off  SenseTotalForce=off  SenseTotalTorque=off  PositionTargetSpecify=on  PositionTargetPriority=High  PositionTargetValue=pi-Rphi230  PositionTargetValueUnits=rad  VelocityTargetSpecify=on  VelocityTargetPriority=High  VelocityTargetValue=0  VelocityTargetValueUnits=rad/s  EquilibriumPosition=0  EquilibriumPositionUnits=deg  SpringStiffness=0  SpringStiffnessUnits=N*m/deg  DampingCoefficient=0  DampingCoefficientUnits=N*m/(deg/s)  LowerLimitSpecify=off  LowerLimitBound=-90  LowerLimitBoundUnits=deg  LowerLimitStiffness=1e4  LowerLimitStiffnessUnits=N*m/deg  LowerLimitDamping=10  LowerLimitDampingUnits=N*m/(deg/s)  LowerLimitTransitionRegionWidth=0.1  LowerLimitTransitionRegionWidthUnits=deg  UpperLimitSpecify=off  UpperLimitBound=90  UpperLimitBoundUnits=deg  UpperLimitStiffness=1e4  UpperLimitStiffnessUnits=N*m/deg  UpperLimitDamping=10  UpperLimitDampingUnits=N*m/(deg/s)  UpperLimitTransitionRegionWidth=0.1  UpperLimitTransitionRegionWidthUnits=deg  TorqueActuationMode=InputTorque  MotionActuationMode=ComputedMotion  SensePosition=on  SenseVelocity=on  SenseAcceleration=off  SenseTorqueForce=off  SenseLowerLimitTorqueForce=off  SenseUpperLimitTorqueForce=off
  Right Foot : Subsystem
  Right Force Plate : Subsystem  TreatAsAtomicUnit=on
  Right Shank : Subsystem
  Right Stance? : Logic  Operator=OR  AllPortsSameDT=off
  Right Thigh Sensor Sheet : Subsystem
  SDelay : TransportDelay  DelayTime=ShortDelay
  SDelay1 : TransportDelay  DelayTime=ShortDelay  InitialOutput=init_theta
  SDelay10 : TransportDelay  DelayTime=ShortDelay  InitialOutput=init_xyzHAT
  SDelay2 : TransportDelay  DelayTime=ShortDelay  InitialOutput=[vx0 0 0]
  SDelay29 : TransportDelay  DelayTime=ShortDelay
  SDelay4 : TransportDelay  DelayTime=ShortDelay
  Selector{,1..3} (4 alike) : Selector  InputPortWidth=3  IndexOptions=Index vector (dialog)  Indices=[1 2]  OutputSizes=1
  Simulink-PS Converter{,1..5} (6 alike) : nesl_utility/Simulink-PS Converter  PhysicalDomain=network_engine_domain  SubClassName=ps_input  LeftPortType=input  RightPortType=output  PseudoPeriodic=off  Frequencies=[]  NoiseDistribution=none  NoiseParameters=[]  Unit=N*m  AffineConversion=off  FilteringAndDerivatives=zero  SimscapeFilterOrder=1  InputFilterTimeConstant=0.001  UdotUserProvided=1
  Solver Configuration : nesl_utility/Solver Configuration  PhysicalDomain=network_engine_domain  SubClassName=solver  LeftPortType=input  RightPortType=generic  Tones=[]  Harmonics=[]  SimulateNoise=off  Profile=off  UseLocalSampling=off  EnableSwitchedLinearOptims=on  FrequencyDomain=off  UseCCode=off  RelTol=0.001  AbsTol=1e-06  MinStep=1e-09  ToWorkspace=off  RevertToSquareIcSolve=off  NumHomotopyIterations=100  PhasorMode=off  PhasorModeNumHarmonics=1  ConsistencySolver=NEWTON_FTOL  IndexReductionMethod=DerivativeReplacement  DoDC=off  ResidualTolerance=1e-09  ConsistencyTolSource=GLOBAL  ConsistencyAbsTol=0.001  ConsistencyRelTol=0.001  ConsistencyTolFactor=0.001  UseLocalSolver=off  LocalSolverChoice=NE_BACKWARD_EULER_ADVANCER  ResolveIndetEquations=on  FunctionEvalNumThread=1  LocalSolverSampleTime=0.001  DoFixedCost=off  MaxNonlinIter=3  MaxModeIter=2  ComputeImpulses=off  ImpulseIterations=2  LinearAlgebra=Sparse  LinearAlgebraNumThread=0  EquationFormulation=NE_TIME_EF  DelaysMemoryBudget=1024  AutomaticFiltering=on  FilteringTimeConstant=0.001  PartitionStorageMethod=AS_NEEDED  PartitionMemoryBudget=1024  PartitionMethod=FAST  MultibodyUseLocalSolver=off  MultibodyLocalSolverChoice=ODE1  MultibodyLocalSolverSampleTime=0.001
  Subsystem1 : Subsystem
  Sum : Sum  Inputs=-+|
  Sum1 : Sum  Inputs=-+|
  Sum{2..5} (4 alike) : Sum  Inputs=++|
  Sum6 : Sum
  Sum7 : Sum
  Sum8 : Sum  Inputs=-+
  Sum9 : Sum  Inputs=+-
  Terminator{,1..5} (6 alike) : Terminator
  Theta : Fcn  Expr=atan2(u(1),u(2))
  Velocity Sensor1 : Subsystem
  Velocity Sensor2 : Subsystem
  Velocity Sensor3 : Subsystem
  World Frame : sm_lib/Frames and Transforms/World Frame
  cnt : Subsystem
  cnt1 : Subsystem
  cnt2 : Subsystem
  cnt3 : Subsystem
  contact information : Subsystem
  contact information1 : Subsystem
  contact information2 : Subsystem
  contact information3 : Subsystem
  dDx : Selector  InputPortWidth=3  IndexOptions=Index vector (dialog)  Indices=[1 2]  OutputSizes=1
  dTheta : Fcn  Expr=( u(2)*u(3) - u(1)*u(4) ) / D1G_HAT^2
  pi{,1..3} (4 alike) : Constant  Value=pi
  pi4 : Constant  Value=pi/2
  pi5 : Constant  Value=pi/2
  plane : sm_lib/Body Elements/Brick Solid  BrickDimensions=[xPla yPla zPla]  BrickDimensionsUnits=m  ExportEntireGeometry=off  InertiaType=CalculateFromGeometry  BasedOnType=Density  Density=1000  DensityUnits=kg/m^3  Mass=1  MassUnits=kg  CenterOfMass=[0 0 0]  CenterOfMassUnits=m  MomentsOfInertia=[1 1 1]  MomentsOfInertiaUnits=kg*m^2  ProductsOfInertia=[1 1 1]  ProductsOfInertiaUnits=kg*m^2  GraphicType=FromGeometry  MarkerShape=Sphere  MarkerSize=10  GraphicVisPropType=SimpleVisualProperties  GraphicDiffuseColor=[0.5 0.5 0.5]  GraphicOpacity=0.5  GraphicSpecularColor=[0.5 0.5 0.5 1.0]  GraphicAmbientColor=[0.15 0.15 0.15 1.0]  GraphicEmissiveColor=[0.0 0.0 0.0 1.0]  GraphicShininess=75  DoExposeReferenceFrame=on  SerializedFrames=<Frames/>
  shift MS to center : sm_lib/Frames and Transforms/Rigid Transform  RotationMethod=StandardAxis  FollAlignAxisA=+X  BaseAlignAxisA=+Y  FollAlignAxisB=+Y  BaseAlignAxisB=+Z  RotationStandardAxis=+Z  RotationAngle=terrain_slope_angle  RotationAngleUnits=rad  RotationArbitraryAxis=[0 0 1]  RotationSequenceAxes=FollowerAxes  RotationSequence=XYX  RotationSequenceAngles=[0 0 0]  RotationSequenceAnglesUnits=deg  RotationMatrix=[1 0 0; 0 1 0; 0 0 1]  Quaternion=[1 0 0 0]  TranslationMethod=Cartesian  TranslationCartesianOffset=[0 0 -D12z_HAT]  TranslationCartesianOffsetUnits=m  TranslationStandardAxis=+Z  TranslationStandardOffset=0  TranslationStandardOffsetUnits=m  TranslationROffset=0  TranslationROffsetUnits=m  TranslationThetaOffset=0  TranslationThetaOffsetUnits=deg  TranslationZOffset=0  TranslationZOffsetUnits=m
  shift plane to center : sm_lib/Frames and Transforms/Rigid Transform  RotationMethod=StandardAxis  FollAlignAxisA=+X  BaseAlignAxisA=+Y  FollAlignAxisB=+Y  BaseAlignAxisB=+Z  RotationStandardAxis=+Z  RotationAngle=terrain_slope_angle  RotationAngleUnits=rad  RotationArbitraryAxis=[0 0 1]  RotationSequenceAxes=FollowerAxes  RotationSequence=XYX  RotationSequenceAngles=[0 0 0]  RotationSequenceAnglesUnits=deg  RotationMatrix=[1 0 0; 0 1 0; 0 0 1]  Quaternion=[1 0 0 0]  TranslationMethod=Cartesian  TranslationCartesianOffset=[xPla/2+xPla_0 -yPla/2+(xPla/2+xPla_0)*tan(terrain_slope_angle) 0]  TranslationCartesianOffsetUnits=m  TranslationStandardAxis=+Z  TranslationStandardOffset=0  TranslationStandardOffsetUnits=m  TranslationROffset=0  TranslationROffsetUnits=m  TranslationThetaOffset=0  TranslationThetaOffsetUnits=deg  TranslationZOffset=0  TranslationZOffsetUnits=m
  tag scope: LBallCnt=global, LGRF=global, LHeelCnt=global, LLLoad=global, LStance=global, Lphi12dphi12=global, Lphi23dphi23=global, Lphi34dphi34=global, RBallCnt=global, RGRF=global, RHeelCnt=global, RLLoad=global, RStance=global, Rphi12dphi12=global, Rphi23dphi23=global, Rphi34dphi34=global, d_LLLoad=global, d_LStance=global, d_RLLoad=global, d_RStance=global, d_dtheta=global, d_theta=global, dd_LStance=global, dd_RStance=global, dd_dtheta=global, dd_dxyzHAT=global, dd_theta=global, dd_xyzHAT=global, dd_xyzLShank1=global, dd_xyzRShank1=global, dtheta=global, dxyzHAT=global, dxyzLHip=global, dxyzRHip=global, theta=global, xyzHAT1=global, xyzHAT2=global, xyzHAT=global, xyzLFoot1=global, xyzLFoot2=global, xyzLHip=global, xyzLShank1=global, xyzLShank2=global, xyzRFoot1=global, xyzRFoot2=global, xyzRHip=global, xyzRShank1=global, xyzRShank2=global, yG_LBall=global, yG_LHeel=global, yG_RBall=global, yG_RHeel=global
  wires:
  Position Sensor6/1(Position) -> SDelay10/1, [xyzHAT]
  Velocity Sensor2/1(Velocity) -> SDelay2/1, [dxyzHAT]
  [LStance] -> Left Force Plate/Enable
  LBall Contact/2(GRF [N N]) -> Left Force Plate/1("GRF_Ball [N N] ")
  LHeel Contact/2(GRF [N N]) -> Left Force Plate/2(GRF_Heel [N N])
  Left Force Plate/1(GRFs) -> [LGRF]
  Left Force Plate/2(COP) -> Terminator1/1
  Velocity Sensor1/1(Velocity) -> [dxyzLHip]
  LHeel Contact/1(Cnt) -> L Heel Skin Load Sensor/1
  L Heel Skin Load Sensor/1 -> [LHeelCnt]
  L Ball Skin Load Sensor/1 -> [LBallCnt]
  LBall Contact/1(Cnt) -> L Ball Skin Load Sensor/1
  L Thigh Displacement  Sensor/1 -> LLoad3/1(dxThigh [m])
  Mux2/1 -> [Lphi34dphi34]
  Mux4/1 -> [Lphi23dphi23]
  Mux6/1 -> [Lphi12dphi12]
  Position Sensor8/1(Position) -> [xyzHAT2]
  Position Sensor5/1(Position) -> [xyzHAT1], [xyzLHip]
  Position Sensor4/1(Position) -> [xyzLShank2]
  Position Sensor3/1(Position) -> LDelay1/1, [xyzLShank1]
  contact information/1(vector) -> Terminator4/1
  contact information1/1(vector) -> Terminator5/1
  LLoad3/1(LLoad [F]) -> SDelay/1, [LLLoad]
  Position Sensor1/1(Position) -> [xyzLFoot1], contact information1/1(point)
  Position Sensor2/1(Position) -> contact information/1(point), [xyzLFoot2]
  PS-Simulink Converter1/1 -> Mux6/2
  PS-Simulink Converter3/1 -> L knee dir/1
  PS-Simulink Converter5/1 -> Mux2/2
  Velocity Sensor3/1(Velocity) -> [dxyzRHip]
  Position Sensor7/1(Position) -> [xyzRHip]
  contact information2/1(vector) -> Terminator3/1
  R Ball Skin Load Sensor/1 -> [RBallCnt]
  Position Sensor12/1(Position) -> [xyzRShank2]
  Position Sensor11/1(Position) -> LDelay2/1, [xyzRShank1]
  RHeel Contact/2(GRF [N N]) -> Right Force Plate/2(GRF_Heel [N N])
  contact information3/1(vector) -> Terminator/1
  Position Sensor9/1(Position) -> [xyzRFoot1], contact information2/1(point)
  Position Sensor10/1(Position) -> [xyzRFoot2], contact information3/1(point)
  Right Force Plate/1(GRFs) -> [RGRF]
  Right Force Plate/2(COP) -> Terminator2/1
  Mux1/1 -> [Rphi34dphi34]
  [RStance] -> Right Force Plate/Enable
  RBall Contact/2(GRF [N N]) -> Right Force Plate/1("GRF_Ball [N N] ")
  RBall Contact/1(Cnt) -> R Ball Skin Load Sensor/1
  R Heel Skin Load Sensor/1 -> [RHeelCnt]
  RHeel Contact/1(Cnt) -> R Heel Skin Load Sensor/1
  LLoad2/1(LLoad [F]) -> SDelay4/1, [RLLoad]
  L knee dir/1 -> Mux4/2
  L knee dir1/1 -> Mux4/1
  PS-Simulink Converter2/1 -> Sum/2
  Sum/1 -> L knee dir1/1
  pi/1 -> Sum/1
  PS-Simulink Converter9/1 -> L knee dir2/1
  Mux3/1 -> [Rphi23dphi23]
  L knee dir2/1 -> Mux3/2
  PS-Simulink Converter8/1 -> Sum1/2
  Sum1/1 -> L knee dir3/1
  L knee dir3/1 -> Mux3/1
  pi1/1 -> Sum1/1
  pi2/1 -> Sum2/1
  PS-Simulink Converter4/1 -> Sum2/2
  PS-Simulink Converter11/1 -> Mux1/2
  PS-Simulink Converter10/1 -> Sum3/2
  Sum3/1 -> Mux1/1
  pi3/1 -> Sum3/1
  pi4/1 -> Sum4/1
  PS-Simulink Converter/1 -> Sum4/2
  Sum4/1 -> Mux6/1
  pi5/1 -> Sum5/1
  PS-Simulink Converter7/1 -> Mux5/2
  Mux5/1 -> [Rphi12dphi12]
  Sum5/1 -> Mux5/1
  PS-Simulink Converter6/1 -> Sum5/2
  Left Thigh Sensor Sheet/1(dx) -> L Thigh Displacement  Sensor/1
  Right Thigh Sensor Sheet/1(dx) -> R Thigh Displacement  Sensor/1
  R Thigh Displacement  Sensor/1 -> LLoad2/1(dxThigh [m])
  [LM12] -> Simulink-PS Converter/1
  [LM23] -> L knee dir6/1
  [LM34] -> Simulink-PS Converter2/1
  [RM23] -> L knee dir7/1
  L knee dir6/1 -> Simulink-PS Converter1/1
  [dxyzLHip] -> Sum7/1
  [dxyzHAT] -> Sum9/1
  " Mean Hip Speed"/1 -> Sum9/2
  "Dx, Dy"/1 -> Mux7/1, Theta/1
  [dxyzRHip] -> Sum7/2
  [xyzRHip] -> Sum6/2
  Mux7/1 -> dTheta/1
  Sum9/1 -> dDx/1
  Sum7/1 -> " Mean Hip Speed"/1
  Mean Hip Position/1 -> Sum8/1
  [xyzLHip] -> Sum6/1
  [xyzHAT] -> Sum8/2
  Sum6/1 -> Mean Hip Position/1
  Sum8/1 -> "Dx, Dy"/1
  dDx/1 -> Mux7/2
  dTheta/1 -> [dtheta], SDelay29/1
  LL Delay4/1 -> [d_dtheta]
  LL Delay1/1 -> [d_theta]
  Theta/1 -> [theta], SDelay1/1
  [LBallCnt] -> Left Stance?/1
  Left Stance?/1 -> [LStance], L Stance afferent delay/1
  [LHeelCnt] -> Left Stance?/2
  L Stance afferent delay/1 -> LL Delay2/1, [d_LStance]
  [RBallCnt] -> Right Stance?/1
  [RHeelCnt] -> Right Stance?/2
  Right Stance?/1 -> [RStance], R Stance afferent delay/1
  R Stance afferent delay/1 -> LL Delay3/1, [d_RStance]
  SDelay/1 -> [d_LLLoad]
  SDelay4/1 -> [d_RLLoad]
  Sum2/1 -> Mux2/1
  [RM12] -> Simulink-PS Converter3/1
  L knee dir7/1 -> Simulink-PS Converter4/1
  [RM34] -> Simulink-PS Converter5/1
  LL Delay2/1 -> [dd_LStance]
  LL Delay3/1 -> [dd_RStance]
  LL Delay5/1 -> [dd_xyzRShank1]
  LDelay2/1 -> LL Delay5/1
  LDelay1/1 -> LL Delay6/1
  LL Delay6/1 -> [dd_xyzLShank1]
  SDelay10/1 -> [dd_xyzHAT]
  SDelay2/1 -> [dd_dxyzHAT]
  SDelay1/1 -> [dd_theta], LL Delay1/1
  SDelay29/1 -> [dd_dtheta], LL Delay4/1
  Selector3/1 -> cnt3/1(Cnt)
  [xyzRFoot2] -> Selector1/1
  cnt3/1(Env) -> [yG_LHeel]
  Selector/1 -> cnt/1(Cnt)
  Selector2/1 -> cnt2/1(Cnt)
  [xyzLFoot1] -> Selector2/1
  Selector1/1 -> cnt1/1(Cnt)
  cnt2/1(Env) -> [yG_LBall]
  [xyzRFoot1] -> Selector/1
  cnt1/1(Env) -> [yG_RHeel]
  cnt/1(Env) -> [yG_RBall]
  [xyzLFoot2] -> Selector3/1
  [yG_RBall] -> RBall Contact/1(Env)
  [yG_RHeel] -> RHeel Contact/1(Env)
  [yG_LHeel] -> LHeel Contact/1(Env)
  [yG_LBall] -> LBall Contact/1(Env)
  connections:
  Left Foot/LConn1 -- Position Sensor2/LConn1 -- LHeel Contact/LConn1
  Left Ankle Joint/LConn1 -- Left Foot/RConn1
  PS-Simulink Converter/LConn1 -- Left Ankle Joint/RConn2
  PS-Simulink Converter1/LConn1 -- Left Ankle Joint/RConn3
  Position Sensor3/LConn1 -- Left Shank2/LConn1 -- Left Ankle Joint/RConn1
  Left Knee Joint1/LConn1 -- Left Shank2/RConn1 -- Position Sensor4/LConn1
  Left Knee Joint1/RConn3 -- PS-Simulink Converter3/LConn1
  Left Knee Joint1/RConn2 -- PS-Simulink Converter2/LConn1
  Left Hip Joint1/RConn3 -- PS-Simulink Converter5/LConn1
  Left Hip Joint1/RConn2 -- PS-Simulink Converter4/LConn1
  Subsystem1/LConn1 -- Position Sensor5/LConn1 -- Velocity Sensor1/LConn1 -- Left Hip Joint1/RConn1
  Position Sensor8/LConn1 -- Subsystem1/RConn2
  Velocity Sensor2/LConn1 -- Position Sensor6/LConn1 -- Subsystem1/RConn1
  Right Knee Joint/LConn1 -- Right Shank/RConn1 -- Position Sensor12/LConn1
  Right Foot/LConn1 -- RHeel Contact/LConn1 -- Position Sensor10/LConn1
  Right Foot/LConn2 -- RBall Contact/LConn1 -- Position Sensor9/LConn1
  Position Sensor11/LConn1 -- Right Ankle Joint/RConn1 -- Right Shank/LConn1
  Right Ankle Joint/LConn1 -- Right Foot/RConn1
  Simulink-PS Converter5/RConn1 -- Right Hip Joint/LConn2
  Right Hip Joint/RConn2 -- PS-Simulink Converter10/LConn1
  Right Hip Joint/RConn3 -- PS-Simulink Converter11/LConn1
  Velocity Sensor3/LConn1 -- Subsystem1/LConn2 -- Position Sensor7/LConn1 -- Right Hip Joint/RConn1
  shift MS to center/LConn1 -- Planar1/RConn1
  Right Knee Joint/RConn2 -- PS-Simulink Converter8/LConn1
  Right Knee Joint/RConn3 -- PS-Simulink Converter9/LConn1
  PS-Simulink Converter6/LConn1 -- Right Ankle Joint/RConn2
  PS-Simulink Converter7/LConn1 -- Right Ankle Joint/RConn3
  Left Thigh Low1/LConn1 -- Right Knee Joint/RConn1
  Left Thigh Sensor Sheet/LConn1 -- Left Thigh Low/RConn1
  Left Thigh High1/RConn1 -- Right Hip Joint/LConn1
  Right Knee Joint/LConn2 -- Simulink-PS Converter4/RConn1
  Simulink-PS Converter3/RConn1 -- Right Ankle Joint/LConn2
  Left Thigh Sensor Sheet/RConn1 -- Left Thigh High/LConn1
  Left Thigh High/RConn1 -- Left Hip Joint1/LConn1
  Left Thigh Low/LConn1 -- Left Knee Joint1/RConn1
  Right Thigh Sensor Sheet/LConn1 -- Left Thigh Low1/RConn1
  Right Thigh Sensor Sheet/RConn1 -- Left Thigh High1/LConn1
  shift plane to center/RConn1 -- plane/RConn1
  Simulink-PS Converter/RConn1 -- Left Ankle Joint/LConn2
  Simulink-PS Converter1/RConn1 -- Left Knee Joint1/LConn2
  Left Hip Joint1/LConn2 -- Simulink-PS Converter2/RConn1
  Left Foot/LConn2 -- Position Sensor1/LConn1 -- shift MS to center/RConn1 -- LBall Contact/LConn1
  Planar1/LConn1 -- Solver Configuration/RConn1 -- World Frame/RConn1 -- shift plane to center/LConn1 -- Mechanism Configuration/RConn1
